simulink model "Fault_RLready_AC_Droop_four_Inverters"  (R2025a)
settings: Solver=ode4  StartTime=0.0  StopTime=15  MaxStep=1e-4  RelTol=1e-3
PreLoadFcn:
  | k_couple = 1;
  | k_power  = 0.0001;
  | k_corr   = 5;
InitFcn:
  | K1=1e-4;
libraries: spsThreePhaseSeriesRLCBranchLib x16, slpidlib x16, spsThreePhaseVIMeasurementLib x12, spsFirstOrderFilterLib x8, spsThreePhaseParallelRLCLoadLib x5, spsDCVoltageSourceLib x4, spsUniversalBridgeLib x4, simulink x4, MGLib x4, spsVoltageMeasurementLib x4, spsThreePhaseBreakerLib x1, spspowerguiLib x1
(part 1 of 4)
settings Model: SimulationMode=accelerator  Creator=Admin  LastModifiedBy=rks9560
settings SolverCC: AlgebraicLoopSolver=TrustRegion
settings OptimizationCC: ReuseModelBlockBuffer=off  EfficientMapNaN2IntZero=off
settings DebuggingCC: UnconnectedInputMsg=warning  UnconnectedOutputMsg=warning  UnconnectedLineMsg=warning  ArithmeticOperatorsInVariantConditions=warning
settings HardwareCC: TargetBitPerPointer=64.0  TargetBitPerSizeT=64.0  TargetBitPerPtrDiffT=64.0  TargetLongLongMode=on  TargetIntDivRoundTo=Zero  TargetEndianess=LittleEndian  TargetWordSize=64.0  TargetHWDeviceType=MATLAB Host  ProdEqTarget=off
settings ModelReferenceCC: EnableRefExpFcnMdlSchedulingChecks=on
settings SFSimCC: SimUseLocalCustomCode=off  CustomCodeUndefinedFunction=UseInterfaceOnly
settings RTWCC: GPUComputeCapability=3.5
settings CodeAppCC: MaxIdLength=128.0
settings GRTTargetCC: TargetLangStandard=C89/C90 (ANSI)  CombineOutputUpdateFcns=off  GRTInterface=on
settings SimscapeCC: SimscapeNormalizeSystem=off

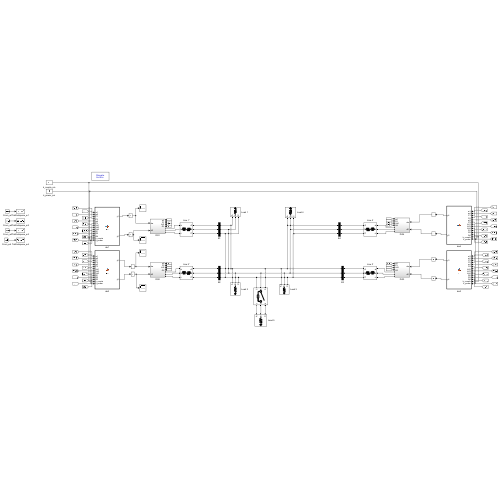
[thumbnail: Simulink's stored preview of the top-level diagram]
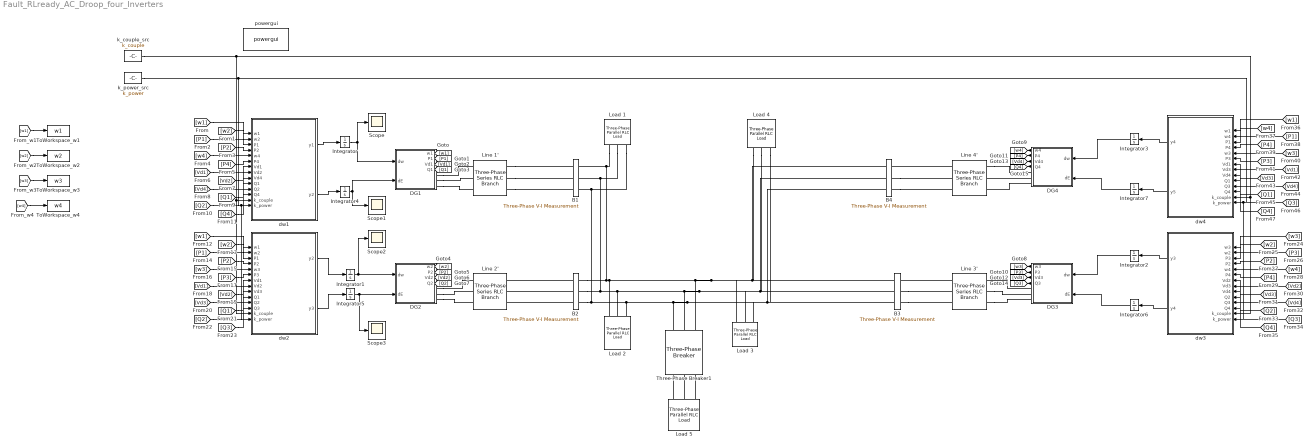
== system Fault_RLready_AC_Droop_four_Inverters ==
  B1 : spsThreePhaseVIMeasurementLib/Three-Phase V-I Measurement  VoltageMeasurement=phase-to-ground  SetLabelV=on  LabelV=VB1  Vpu=off  VpuLL=off  CurrentMeasurement=yes  SetLabelI=on  LabelI=IB1  Ipu=off  Pbase=100e6  Vbase=500e3  OutputType=Complex  PhasorSimulation=off  PSBequivalent=0
  B2 : spsThreePhaseVIMeasurementLib/Three-Phase V-I Measurement  VoltageMeasurement=phase-to-ground  SetLabelV=on  LabelV=VB2  Vpu=off  VpuLL=off  CurrentMeasurement=yes  SetLabelI=on  LabelI=IB2  Ipu=off  Pbase=100e6  Vbase=500e3  OutputType=Complex  PhasorSimulation=off  PSBequivalent=0
  B3 : spsThreePhaseVIMeasurementLib/Three-Phase V-I Measurement  VoltageMeasurement=phase-to-ground  SetLabelV=on  LabelV=VB3  Vpu=off  VpuLL=off  CurrentMeasurement=yes  SetLabelI=on  LabelI=IB3  Ipu=off  Pbase=100e6  Vbase=500e3  OutputType=Complex  PhasorSimulation=off  PSBequivalent=0
  B4 : spsThreePhaseVIMeasurementLib/Three-Phase V-I Measurement  VoltageMeasurement=phase-to-ground  SetLabelV=on  LabelV=VB4  Vpu=off  VpuLL=off  CurrentMeasurement=yes  SetLabelI=on  LabelI=IB4  Ipu=off  Pbase=100e6  Vbase=500e3  OutputType=Complex  PhasorSimulation=off  PSBequivalent=0
  DG1 : Subsystem
  DG2 : Subsystem
  DG3 : Subsystem
  DG4 : Subsystem
  Integrator{,1..7} (8 alike) : Integrator
  Line 1' : spsThreePhaseSeriesRLCBranchLib/Three-Phase Series RLC Branch  LConnTagsString=A|B|C  RConnTagsString=A|B|C  BranchType=RL  Resistance=0.07  Inductance=0.05e-2  Capacitance=1e-6  Measurements=None
  Line 2' : spsThreePhaseSeriesRLCBranchLib/Three-Phase Series RLC Branch  LConnTagsString=A|B|C  RConnTagsString=A|B|C  BranchType=RL  Resistance=0.07  Inductance=0.05e-2  Capacitance=1e-6  Measurements=None
  Line 3' : spsThreePhaseSeriesRLCBranchLib/Three-Phase Series RLC Branch  LConnTagsString=A|B|C  RConnTagsString=A|B|C  BranchType=RL  Resistance=0.01  Inductance=0.05e-2  Capacitance=1e-6  Measurements=None
  Line 4' : spsThreePhaseSeriesRLCBranchLib/Three-Phase Series RLC Branch  LConnTagsString=A|B|C  RConnTagsString=A|B|C  BranchType=RL  Resistance=0.07  Inductance=0.05e-2  Capacitance=1e-6  Measurements=None
  Load {1..4} (4 alike) : spsThreePhaseParallelRLCLoadLib/Three-Phase Parallel RLC Load  LConnTagsString=A|B|C  Configuration=Y (grounded)  NominalVoltage=415  Vabc=[1e3 1e3 1e3]  Vabcp=[1e3 1e3 1e3]  NominalFrequency=60  UnbalancedPower=off  ActivePower=5e3  InductivePower=0  CapacitivePower=0  Pabc=[10e3 9e3 11e3]  QLabc=[100 90 110]  QCabc=[100 90 110]  Pabcp=[10e3 9e3 11e3]  QLabcp=[100 90 110]  QCabcp=[100 90 110]  Measurements=None  LoadType=constant PQ
  Load 5 : spsThreePhaseParallelRLCLoadLib/Three-Phase Parallel RLC Load  LConnTagsString=A|B|C  Configuration=Y (grounded)  NominalVoltage=415  Vabc=[1e3 1e3 1e3]  Vabcp=[1e3 1e3 1e3]  NominalFrequency=60  UnbalancedPower=off  ActivePower=20e3  InductivePower=0  CapacitivePower=0  Pabc=[10e3 9e3 11e3]  QLabc=[100 90 110]  QCabc=[100 90 110]  Pabcp=[10e3 9e3 11e3]  QLabcp=[100 90 110]  QCabcp=[100 90 110]  Measurements=None  LoadType=constant PQ
  Scope{,1..3} (4 alike) : Scope
      Scope settings: ActiveDisplayYMinimum=-117.83448  ActiveDisplayYMaximum=1060.51036
      Scope1 settings: ActiveDisplayYMinimum=-75.78712  ActiveDisplayYMaximum=9.50958  DataLoggingVariableName=ScopeData2
      Scope2 settings: ActiveDisplayYMinimum=-0.02486  ActiveDisplayYMaximum=0.2237  DataLoggingVariableName=ScopeData3
      Scope3 settings: ActiveDisplayYMinimum=-0.00731  ActiveDisplayYMaximum=0.06583  DataLoggingVariableName=ScopeData4
  Three-Phase Breaker1 : spsThreePhaseBreakerLib/Three-Phase Breaker  InitialState=open  SwitchA=on  SwitchB=on  SwitchC=on  SwitchTimes=[6]  External=off  BreakerResistance=0.01  SnubberResistance=1e6  SnubberCapacitance=inf  Measurements=None
  ToWorkspace_w1 : ToWorkspace  VariableName=w1  SaveFormat=Structure With Time  SampleTime=-1
  ToWorkspace_w2 : ToWorkspace  VariableName=w2  SaveFormat=Structure With Time  SampleTime=-1
  ToWorkspace_w3 : ToWorkspace  VariableName=w3  SaveFormat=Structure With Time  SampleTime=-1
  ToWorkspace_w4 : ToWorkspace  VariableName=w4  SaveFormat=Structure With Time  SampleTime=-1
  dw1 : MATLAB Function  TreatAsAtomicUnit=on
  dw2 : MATLAB Function  TreatAsAtomicUnit=on
  dw3 : MATLAB Function  TreatAsAtomicUnit=on
  dw4 : MATLAB Function  TreatAsAtomicUnit=on
  k_couple_src : Constant  Value=k_couple
  k_power_src : Constant  Value=k_power
  powergui : spspowerguiLib/powergui  Priority=1  SimulationMode=Discrete  SampleTime=0.2e-5  frequency=60  Iterations=50  frequencyindice=0  Pbase=100e6  ErrMax=1e-4  UnitsV=kV  UnitsW=MW  buscounter=0  FunctionMessages=off  echomessages=off  EnableUseOfTLC=off  CurrentSourceSwitches=off  DisableSnubberDevices=off  DisableRonSwitches=off  DisableVfSwitches=off  DisplayEquations=off  AutomaticDiscreteSolvers=off  SolverType=Tustin/Backward Euler (TBE)  Interpol=off  ExternalGateDelay=off  methode=off  Ts=100  x0status=blocks  SPID=off  SwTol=0  HookPort=off  NonlinearTolerance=1e-4  nMaxIteration=100  ContinueOnMaxIteration=off  RestoreLinks=warning  ResistiveCurrentMeasurement=off  Frange=[0:2:500]  Ylog=off  Xlog=on  ShowGrid=off  save=off  variable=ZData  structure=0  ZoomFFT=off  StartTime=0.0  cycles=1  DisplayStyle=1  fundamental=60  FreqAxis=off  MaxFrequency=1000  frequencyindicesteady=1  RmsSteady=1  display=off
  wires:
  Integrator2/1 -> DG3/1(dw)
  Integrator3/1 -> DG4/1(dw)
  dw1/1(y1) -> Integrator/1
  dw2/1(y2) -> Integrator1/1
  dw4/1(y4) -> Integrator3/1
  dw3/1(y3) -> Integrator2/1
  dw1/2(y2) -> Integrator4/1
  dw2/2(y3) -> Integrator5/1
  dw3/2(y4) -> Integrator6/1
  Integrator6/1 -> DG3/2(dE)
  dw4/2(y5) -> Integrator7/1
  Integrator7/1 -> DG4/2(dE)
  DG4/3(Vd4) -> [Vd4]
  DG1/1(w1) -> [w1]
  DG1/2(P1) -> [P1]
  DG1/3(Vd1) -> [Vd1]
  DG1/4(Q1) -> [Q1]
  DG2/1(w2) -> [w2]
  DG2/2(P2) -> [P2]
  DG2/3(Vd2) -> [Vd2]
  DG2/4(Q2) -> [Q2]
  DG3/1(w3) -> [w3]
  DG4/1(w4) -> [w4]
  DG3/2(P3) -> [P3]
  DG4/2(P4) -> [P4]
  DG3/3(Vd3) -> [Vd3]
  DG3/4(Q3) -> [Q3]
  DG4/4(Q4) -> [Q4]
  Integrator/1 -> DG1/1(dw), Scope/1
  Integrator4/1 -> DG1/2(dE), Scope1/1
  Integrator1/1 -> DG2/1(dw), Scope2/1
  Integrator5/1 -> Scope3/1, DG2/2(dE)
  [w1] -> dw1/1(w1)
  [w2] -> dw1/2(w2)
  [P1] -> dw1/3(P1)
  [P2] -> dw1/4(P2)
  [w4] -> dw1/5(w4)
  [P4] -> dw1/6(P4)
  [Vd1] -> dw1/7(Vd1)
  [Vd2] -> dw1/8(Vd2)
  [Vd4] -> dw1/9(Vd4)
  [Q1] -> dw1/10(Q1)
  [Q2] -> dw1/11(Q2)
  [Q4] -> dw1/12(Q4)
  [w1] -> dw2/1(w1)
  [w2] -> dw2/2(w2)
  [P1] -> dw2/3(P1)
  [P2] -> dw2/4(P2)
  [w3] -> dw2/5(w3)
  [P3] -> dw2/6(P3)
  [Vd1] -> dw2/7(Vd1)
  [Vd2] -> dw2/8(Vd2)
  [Vd3] -> dw2/9(Vd3)
  [Q1] -> dw2/10(Q1)
  [Q2] -> dw2/11(Q2)
  [Q3] -> dw2/12(Q3)
  [w1] -> dw4/1(w1)
  [w4] -> dw4/2(w4)
  [P1] -> dw4/3(P1)
  [P4] -> dw4/4(P4)
  [w3] -> dw4/5(w3)
  [P3] -> dw4/6(P3)
  [Vd1] -> dw4/7(Vd1)
  [Vd3] -> dw4/8(Vd3)
  [Vd4] -> dw4/9(Vd4)
  [Q1] -> dw4/10(Q1)
  [Q3] -> dw4/11(Q3)
  [Q4] -> dw4/12(Q4)
  [w3] -> dw3/1(w3)
  [w2] -> dw3/2(w2)
  [P3] -> dw3/3(P3)
  [P2] -> dw3/4(P2)
  [w4] -> dw3/5(w4)
  [P4] -> dw3/6(P4)
  [Vd2] -> dw3/7(Vd2)
  [Vd3] -> dw3/8(Vd3)
  [Vd4] -> dw3/9(Vd4)
  [Q2] -> dw3/10(Q2)
  [Q3] -> dw3/11(Q3)
  [Q4] -> dw3/12(Q4)
  k_couple_src/1 -> dw4/13(k_couple), dw3/13(k_couple), dw1/13(k_couple), dw2/13(k_couple)
  k_power_src/1 -> dw3/14(k_power), dw4/14(k_power), dw1/14(k_power), dw2/14(k_power)
  [w1] -> ToWorkspace_w1/1
  [w2] -> ToWorkspace_w2/1
  [w3] -> ToWorkspace_w3/1
  [w4] -> ToWorkspace_w4/1
  connections:
  Line 1'/LConn3 -- B1/LConn3
  Line 1'/LConn1 -- B1/LConn1
  Line 1'/LConn2 -- B1/LConn2
  B2/LConn1 -- Line 2'/LConn1
  B2/LConn2 -- Line 2'/LConn2
  B2/LConn3 -- Line 2'/LConn3
  Line 3'/LConn1 -- B3/LConn1
  B3/LConn2 -- Line 3'/LConn2
  B3/LConn3 -- Line 3'/LConn3
  Line 4'/LConn1 -- B4/LConn1
  B4/LConn2 -- Line 4'/LConn2
  B4/LConn3 -- Line 4'/LConn3
  B2/RConn1 -- Three-Phase Breaker1/LConn1 -- B3/RConn1 -- B4/RConn1 -- Load 4/LConn1 -- Load 3/LConn1 -- Load 2/LConn1 -- Load 1/LConn1 -- B1/RConn1
  B2/RConn2 -- Three-Phase Breaker1/LConn2 -- B3/RConn2 -- B4/RConn2 -- Load 4/LConn2 -- Load 3/LConn2 -- Load 2/LConn2 -- Load 1/LConn2 -- B1/RConn2
  B2/RConn3 -- Three-Phase Breaker1/LConn3 -- B3/RConn3 -- B4/RConn3 -- Load 4/LConn3 -- Load 3/LConn3 -- Load 2/LConn3 -- Load 1/LConn3 -- B1/RConn3
  DG1/RConn1 -- Line 1'/RConn1
  DG1/RConn2 -- Line 1'/RConn2
  DG1/RConn3 -- Line 1'/RConn3
  DG2/RConn1 -- Line 2'/RConn1
  DG2/RConn2 -- Line 2'/RConn2
  DG2/RConn3 -- Line 2'/RConn3
  DG3/RConn1 -- Line 3'/RConn1
  Line 3'/RConn2 -- DG3/RConn2
  Line 3'/RConn3 -- DG3/RConn3
  Line 4'/RConn1 -- DG4/RConn1
  DG4/RConn2 -- Line 4'/RConn2
  DG4/RConn3 -- Line 4'/RConn3
  Load 5/LConn1 -- Three-Phase Breaker1/RConn3
  Load 5/LConn2 -- Three-Phase Breaker1/RConn2
  Load 5/LConn3 -- Three-Phase Breaker1/RConn1

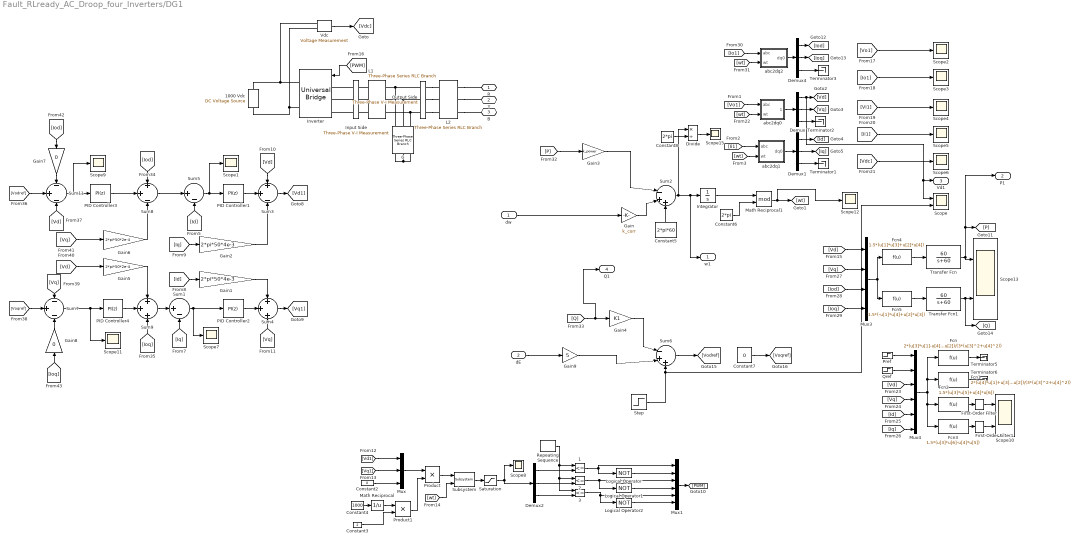
== system Fault_RLready_AC_Droop_four_Inverters/DG1 ==
  dw : Inport
  dE : Inport  Port=2
  1 : RelationalOperator  Operator=<=  OutDataTypeStr=boolean  RndMeth=Simplest  InputSameDT=off
  1000 Vdc : spsDCVoltageSourceLib/DC Voltage Source  Amplitude=1000  Measurements=None
  2 : RelationalOperator  Operator=<=  OutDataTypeStr=boolean  RndMeth=Simplest  InputSameDT=off
  3 : RelationalOperator  Operator=<=  OutDataTypeStr=boolean  RndMeth=Simplest  InputSameDT=off
  C : spsThreePhaseSeriesRLCBranchLib/Three-Phase Series RLC Branch  LConnTagsString=A|B|C  RConnTagsString=A|B|C  BranchType=RC  Resistance=5  Inductance=1e-3  Capacitance=2e-4  Measurements=None
  Constant2 : Constant  Value=0
  Constant3 : Constant  Value=2
  Constant4 : Constant  Value=1000
  Constant5 : Constant  Value=2*pi*60
  Constant6 : Constant  Value=2*pi
  Constant7 : Constant  Value=0
  Constant8 : Constant  Value=2*pi
  Demux{,1..2,4} (4 alike) : Demux  Outputs=3
  Divide : Product  Inputs=*/
  Fcn : Fcn  Expr=2*(u[3]*u[1]-u[4]*u[2])/(3*(u[3]^2+u[4]^2))
  Fcn1 : Fcn  Expr=2*(u[4]*u[1]+u[3]*u[2])/(3*(u[3]^2+u[4]^2))
  Fcn2 : Fcn  Expr=1.5*(u[3]*u[5]+u[4]*u[6])
  Fcn3 : Fcn  Expr=1.5*(u[3]*u[6]-u[4]*u[5])
  Fcn4 : Fcn  Expr=1.5*(u[1]*u[3]+u[2]*u[4])
  Fcn5 : Fcn  Expr=1.5*(-u[1]*u[4]+u[2]*u[3])
  First-Order Filter : spsFirstOrderFilterLib/First-Order Filter  FilterType=Lowpass  Tc=0.03  Ts=0  Initialize=on  Vac_Init=[0, 0, 60]  Vdc_Init=0  PlotResponse=off  FreqRange="[0,  200,  1]"
  First-Order Filter1 : spsFirstOrderFilterLib/First-Order Filter  FilterType=Lowpass  Tc=0.03  Ts=0  Initialize=on  Vac_Init=[0, 0, 60]  Vdc_Init=0  PlotResponse=off  FreqRange="[0,  200,  1]"
  Gain : Gain  Gain=k_corr
  Gain1 : Gain  Gain=2*pi*50*4e-3
  Gain2 : Gain  Gain=2*pi*50*4e-3
  Gain3 : Gain  Gain=k_power
  Gain4 : Gain  Gain=K1
  Gain5 : Gain  Gain=2*pi*50*2e-4
  Gain6 : Gain  Gain=2*pi*50*2e-4
  Gain7 : Gain  Gain=0
  Gain8 : Gain  Gain=0
  Gain9 : Gain  Gain=5
  Input Side : spsThreePhaseVIMeasurementLib/Three-Phase V-I Measurement  VoltageMeasurement=phase-to-ground  SetLabelV=on  LabelV=Vi1  Vpu=off  VpuLL=off  CurrentMeasurement=yes  SetLabelI=on  LabelI=Ii1  Ipu=off  Pbase=100e6  Vbase=500e3  OutputType=Complex  PhasorSimulation=off  PSBequivalent=0
  Integrator : Integrator
  Inverter : spsUniversalBridgeLib/Universal Bridge  Arms=3  SnubberResistance=1e5  SnubberCapacitance=inf  Device=Ideal Switches  Ron=1e-3  Lon=0  ForwardVoltages="[  0  0  ]"  ForwardVoltage=0  GTOparameters=[ 10e-6 , 20e-6 ]  IGBTparameters=[ 1e-6 , 2e-6 ]  Measurements=None  Measurements_2=None  converterType=Rectifier
  L1 : spsThreePhaseSeriesRLCBranchLib/Three-Phase Series RLC Branch  LConnTagsString=A|B|C  RConnTagsString=A|B|C  BranchType=RL  Resistance=0.1  Inductance=4e-3  Capacitance=1e-6  Measurements=None
  L2 : spsThreePhaseSeriesRLCBranchLib/Three-Phase Series RLC Branch  LConnTagsString=A|B|C  RConnTagsString=A|B|C  BranchType=RL  Resistance=0.03  Inductance=1e-3  Capacitance=1e-6  Measurements=None
  Logical Operator : Logic  Operator=NOT  IconShape=distinctive  AllPortsSameDT=off  OutDataTypeStr=boolean
  Logical Operator1 : Logic  Operator=NOT  IconShape=distinctive  AllPortsSameDT=off  OutDataTypeStr=boolean
  Logical Operator2 : Logic  Operator=NOT  IconShape=distinctive  AllPortsSameDT=off  OutDataTypeStr=boolean
  Math Reciprocal : Math  Operator=reciprocal  SignedPower=on
  Math Reciprocal1 : Math  Operator=mod  SignedPower=on
  Mux : Mux  Inputs=3
  Mux1 : Mux  Inputs=6
  Mux3 : Mux
  Mux4 : Mux  Inputs=6
  Output Side : spsThreePhaseVIMeasurementLib/Three-Phase V-I Measurement  VoltageMeasurement=phase-to-ground  SetLabelV=on  LabelV=Vo1  Vpu=off  VpuLL=off  CurrentMeasurement=yes  SetLabelI=on  LabelI=Io1  Ipu=off  Pbase=100e6  Vbase=500e3  OutputType=Complex  PhasorSimulation=off  PSBequivalent=0
  PID Controller1 : slpidlib/PID Controller  Controller=PI  Form=Parallel  TimeDomain=Discrete-time  UseExternalTs=off  SampleTime=-1  IntegratorMethod=Forward Euler  FilterMethod=Forward Euler  ControllerParametersSource=internal  P=4e-3/1e-4  I=0.1/1e-4  UseKiTs=off  D=0  UseExternalDerivativeSource=off  N=100  UseFilter=on  TunerSelectOption=Transfer Function Based (PID Tuner App)  InitialConditionSource=internal  InitialConditionForIntegrator=0  InitialConditionForFilter=0  DifferentiatorICPrevScaledInput=0  ExternalReset=none  TrackingMode=off  Kt=1  LimitOutput=off  SatLimitsSource=internal  UpperSaturationLimit=inf  LowerSaturationLimit=-inf  LinearizeAsGain=on  AntiWindupMode=none  Kb=1  LimitIntegrator=off  UpperIntegratorSaturationLimit=inf  LowerIntegratorSaturationLimit=-inf  POutMin=[]  POutMax=[]  IOutMin=[]  IOutMax=[]  DOutMin=[]  DOutMax=[]  NOutMin=[]  NOutMax=[]  SumOutMin=[]  SumOutMax=[]  SaturationOutMin=[]  SaturationOutMax=[]  PParamMin=[]  PParamMax=[]  IParamMin=[]  IParamMax=[]  DParamMin=[]  DParamMax=[]  NParamMin=[]  NParamMax=[]  KbParamMin=[]  KbParamMax=[]  KtParamMin=[]  KtParamMax=[]  KbOutMin=[]  KbOutMax=[]  KtOutMin=[]  KtOutMax=[]  IntegratorOutMin=[]  IntegratorOutMax=[]  FilterOutMin=[]  FilterOutMax=[]  SumI1OutMin=[]  SumI1OutMax=[]  SumI2OutMin=[]  SumI2OutMax=[]  SumI3OutMin=[]  SumI3OutMax=[]  SumI4OutMin=[]  SumI4OutMax=[]  SumDOutMin=[]  SumDOutMax=[]  DifferentiatorOutMin=[]  DifferentiatorOutMax=[]  FilterDiffOutCoefMin=[]  FilterDiffOutCoefMax=[]  ReciprocalOutMin=[]  ReciprocalOutMax=[]  SumDenOutMin=[]  SumDenOutMax=[]  SumNumOutMin=[]  SumNumOutMax=[]  DivideOutMin=[]  DivideOutMax=[]  UdiffTsProdOutMin=[]  UdiffTsProdOutMax=[]  NTsProdOutMin=[]  NTsProdOutMax=[]  UintegralTsProdOutMin=[]  UintegralTsProdOutMax=[]  UngainTsProdOutMin=[]  UngainTsProdOutMax=[]  ClampingZeroOutDataTypeStr=Inherit: Inherit via back propagation  ClampingZeroOutMin=[]  ClampingZeroOutMax=[]  FilterDenConstantOutDataTypeStr=Inherit: Inherit via back propagation  FilterDenConstantOutMin=[]  FilterDenConstantOutMax=[]  PCopyOutDataTypeStr=Inherit: Inherit via back propagation  PCopyOutMin=[]  PCopyOutMax=[]  NCopyOutDataTypeStr=Inherit: Inherit via back propagation  NCopyOutMin=[]  NCopyOutMax=[]  IntegratorContinuousStateAttributes=''  IntegratorStateMustResolveToSignalObject=off  IntegratorRTWStateStorageClass=Auto  FilterContinuousStateAttributes=''  FilterStateMustResolveToSignalObject=off  FilterRTWStateStorageClass=Auto  ParallelPVariant=InternalParameters  IdealPVariant=Disabled  IVariant=InternalParameters  DVariant=Disabled  IntegratorVariant=Discrete  SatVariant=Disabled  AWVariant=Passthrough  PCopyVariant=Disabled  TRVariant=Disabled  FdbkBlocksVariant=Forward  IdealPFdbkVariant=Disabled  SatFdbkVariant=Disabled  DerivativeFilterVariant=Disabled  NVariant=Disabled  NCopyVariant=Disabled_SignalSpec  FilterICVariant=Disabled  IntegratorICVariant=InternalICs  ExternalResetVariant=Disabled  TRSumVariant=Passthrough  SumFdbkVariant=Disabled  SumVariant=Sum_PI  TsampFilterVariant=InternalTs  TsampNgainVariant=Passthrough  TsampIntegralVariant=Disabled_SignalSpec  ExternalSaturationOutDataTypeStr=Inherit: Same as second input  DerivativeSourceVariant=Disabled  PreIntVariant=InternalPreInt
  PID Controller2 : slpidlib/PID Controller  Controller=PI  Form=Parallel  TimeDomain=Discrete-time  UseExternalTs=off  SampleTime=-1  IntegratorMethod=Forward Euler  FilterMethod=Forward Euler  ControllerParametersSource=internal  P=4e-3/1e-4  I=0.1/1e-4  UseKiTs=off  D=0  UseExternalDerivativeSource=off  N=100  UseFilter=on  TunerSelectOption=Transfer Function Based (PID Tuner App)  InitialConditionSource=internal  InitialConditionForIntegrator=0  InitialConditionForFilter=0  DifferentiatorICPrevScaledInput=0  ExternalReset=none  TrackingMode=off  Kt=1  LimitOutput=off  SatLimitsSource=internal  UpperSaturationLimit=inf  LowerSaturationLimit=-inf  LinearizeAsGain=on  AntiWindupMode=none  Kb=1  LimitIntegrator=off  UpperIntegratorSaturationLimit=inf  LowerIntegratorSaturationLimit=-inf  POutMin=[]  POutMax=[]  IOutMin=[]  IOutMax=[]  DOutMin=[]  DOutMax=[]  NOutMin=[]  NOutMax=[]  SumOutMin=[]  SumOutMax=[]  SaturationOutMin=[]  SaturationOutMax=[]  PParamMin=[]  PParamMax=[]  IParamMin=[]  IParamMax=[]  DParamMin=[]  DParamMax=[]  NParamMin=[]  NParamMax=[]  KbParamMin=[]  KbParamMax=[]  KtParamMin=[]  KtParamMax=[]  KbOutMin=[]  KbOutMax=[]  KtOutMin=[]  KtOutMax=[]  IntegratorOutMin=[]  IntegratorOutMax=[]  FilterOutMin=[]  FilterOutMax=[]  SumI1OutMin=[]  SumI1OutMax=[]  SumI2OutMin=[]  SumI2OutMax=[]  SumI3OutMin=[]  SumI3OutMax=[]  SumI4OutMin=[]  SumI4OutMax=[]  SumDOutMin=[]  SumDOutMax=[]  DifferentiatorOutMin=[]  DifferentiatorOutMax=[]  FilterDiffOutCoefMin=[]  FilterDiffOutCoefMax=[]  ReciprocalOutMin=[]  ReciprocalOutMax=[]  SumDenOutMin=[]  SumDenOutMax=[]  SumNumOutMin=[]  SumNumOutMax=[]  DivideOutMin=[]  DivideOutMax=[]  UdiffTsProdOutMin=[]  UdiffTsProdOutMax=[]  NTsProdOutMin=[]  NTsProdOutMax=[]  UintegralTsProdOutMin=[]  UintegralTsProdOutMax=[]  UngainTsProdOutMin=[]  UngainTsProdOutMax=[]  ClampingZeroOutDataTypeStr=Inherit: Inherit via back propagation  ClampingZeroOutMin=[]  ClampingZeroOutMax=[]  FilterDenConstantOutDataTypeStr=Inherit: Inherit via back propagation  FilterDenConstantOutMin=[]  FilterDenConstantOutMax=[]  PCopyOutDataTypeStr=Inherit: Inherit via back propagation  PCopyOutMin=[]  PCopyOutMax=[]  NCopyOutDataTypeStr=Inherit: Inherit via back propagation  NCopyOutMin=[]  NCopyOutMax=[]  IntegratorContinuousStateAttributes=''  IntegratorStateMustResolveToSignalObject=off  IntegratorRTWStateStorageClass=Auto  FilterContinuousStateAttributes=''  FilterStateMustResolveToSignalObject=off  FilterRTWStateStorageClass=Auto  ParallelPVariant=InternalParameters  IdealPVariant=Disabled  IVariant=InternalParameters  DVariant=Disabled  IntegratorVariant=Discrete  SatVariant=Disabled  AWVariant=Passthrough  PCopyVariant=Disabled  TRVariant=Disabled  FdbkBlocksVariant=Forward  IdealPFdbkVariant=Disabled  SatFdbkVariant=Disabled  DerivativeFilterVariant=Disabled  NVariant=Disabled  NCopyVariant=Disabled_SignalSpec  FilterICVariant=Disabled  IntegratorICVariant=InternalICs  ExternalResetVariant=Disabled  TRSumVariant=Passthrough  SumFdbkVariant=Disabled  SumVariant=Sum_PI  TsampFilterVariant=InternalTs  TsampNgainVariant=Passthrough  TsampIntegralVariant=Disabled_SignalSpec  ExternalSaturationOutDataTypeStr=Inherit: Same as second input  DerivativeSourceVariant=Disabled  PreIntVariant=InternalPreInt
  PID Controller3 : slpidlib/PID Controller  Controller=PI  Form=Parallel  TimeDomain=Discrete-time  UseExternalTs=off  SampleTime=-1  IntegratorMethod=Forward Euler  FilterMethod=Forward Euler  ControllerParametersSource=internal  P=2e-4/1e-3  I=5/1e-3  UseKiTs=off  D=0  UseExternalDerivativeSource=off  N=100  UseFilter=on  TunerSelectOption=Transfer Function Based (PID Tuner App)  InitialConditionSource=internal  InitialConditionForIntegrator=0  InitialConditionForFilter=0  DifferentiatorICPrevScaledInput=0  ExternalReset=none  TrackingMode=off  Kt=1  LimitOutput=off  SatLimitsSource=internal  UpperSaturationLimit=40  LowerSaturationLimit=-40  LinearizeAsGain=on  AntiWindupMode=back-calculation  Kb=1  LimitIntegrator=off  UpperIntegratorSaturationLimit=inf  LowerIntegratorSaturationLimit=-inf  POutMin=[]  POutMax=[]  IOutMin=[]  IOutMax=[]  DOutMin=[]  DOutMax=[]  NOutMin=[]  NOutMax=[]  SumOutMin=[]  SumOutMax=[]  SaturationOutMin=[]  SaturationOutMax=[]  PParamMin=[]  PParamMax=[]  IParamMin=[]  IParamMax=[]  DParamMin=[]  DParamMax=[]  NParamMin=[]  NParamMax=[]  KbParamMin=[]  KbParamMax=[]  KtParamMin=[]  KtParamMax=[]  KbOutMin=[]  KbOutMax=[]  KtOutMin=[]  KtOutMax=[]  IntegratorOutMin=[]  IntegratorOutMax=[]  FilterOutMin=[]  FilterOutMax=[]  SumI1OutMin=[]  SumI1OutMax=[]  SumI2OutMin=[]  SumI2OutMax=[]  SumI3OutMin=[]  SumI3OutMax=[]  SumI4OutMin=[]  SumI4OutMax=[]  SumDOutMin=[]  SumDOutMax=[]  DifferentiatorOutMin=[]  DifferentiatorOutMax=[]  FilterDiffOutCoefMin=[]  FilterDiffOutCoefMax=[]  ReciprocalOutMin=[]  ReciprocalOutMax=[]  SumDenOutMin=[]  SumDenOutMax=[]  SumNumOutMin=[]  SumNumOutMax=[]  DivideOutMin=[]  DivideOutMax=[]  UdiffTsProdOutMin=[]  UdiffTsProdOutMax=[]  NTsProdOutMin=[]  NTsProdOutMax=[]  UintegralTsProdOutMin=[]  UintegralTsProdOutMax=[]  UngainTsProdOutMin=[]  UngainTsProdOutMax=[]  ClampingZeroOutDataTypeStr=Inherit: Inherit via back propagation  ClampingZeroOutMin=[]  ClampingZeroOutMax=[]  FilterDenConstantOutDataTypeStr=Inherit: Inherit via back propagation  FilterDenConstantOutMin=[]  FilterDenConstantOutMax=[]  PCopyOutDataTypeStr=Inherit: Inherit via back propagation  PCopyOutMin=[]  PCopyOutMax=[]  NCopyOutDataTypeStr=Inherit: Inherit via back propagation  NCopyOutMin=[]  NCopyOutMax=[]  IntegratorContinuousStateAttributes=''  IntegratorStateMustResolveToSignalObject=off  IntegratorRTWStateStorageClass=Auto  FilterContinuousStateAttributes=''  FilterStateMustResolveToSignalObject=off  FilterRTWStateStorageClass=Auto  ParallelPVariant=InternalParameters  IdealPVariant=Disabled  IVariant=InternalParameters  DVariant=Disabled  IntegratorVariant=Discrete  SatVariant=Disabled  AWVariant=Passthrough  PCopyVariant=Disabled  TRVariant=Disabled  FdbkBlocksVariant=Forward  IdealPFdbkVariant=Disabled  SatFdbkVariant=Disabled  DerivativeFilterVariant=Disabled  NVariant=Disabled  NCopyVariant=Disabled_SignalSpec  FilterICVariant=Disabled  IntegratorICVariant=InternalICs  ExternalResetVariant=Disabled  TRSumVariant=Passthrough  SumFdbkVariant=Disabled  SumVariant=Sum_PI  TsampFilterVariant=InternalTs  TsampNgainVariant=Passthrough  TsampIntegralVariant=Disabled_SignalSpec  ExternalSaturationOutDataTypeStr=Inherit: Same as second input  DerivativeSourceVariant=Disabled  PreIntVariant=InternalPreInt
  PID Controller4 : slpidlib/PID Controller  Controller=PI  Form=Parallel  TimeDomain=Discrete-time  UseExternalTs=off  SampleTime=-1  IntegratorMethod=Forward Euler  FilterMethod=Forward Euler  ControllerParametersSource=internal  P=2e-4/1e-3  I=5/1e-3  UseKiTs=off  D=0  UseExternalDerivativeSource=off  N=100  UseFilter=on  TunerSelectOption=Transfer Function Based (PID Tuner App)  InitialConditionSource=internal  InitialConditionForIntegrator=0  InitialConditionForFilter=0  DifferentiatorICPrevScaledInput=0  ExternalReset=none  TrackingMode=off  Kt=1  LimitOutput=off  SatLimitsSource=internal  UpperSaturationLimit=40  LowerSaturationLimit=-40  LinearizeAsGain=on  AntiWindupMode=back-calculation  Kb=1  LimitIntegrator=off  UpperIntegratorSaturationLimit=inf  LowerIntegratorSaturationLimit=-inf  POutMin=[]  POutMax=[]  IOutMin=[]  IOutMax=[]  DOutMin=[]  DOutMax=[]  NOutMin=[]  NOutMax=[]  SumOutMin=[]  SumOutMax=[]  SaturationOutMin=[]  SaturationOutMax=[]  PParamMin=[]  PParamMax=[]  IParamMin=[]  IParamMax=[]  DParamMin=[]  DParamMax=[]  NParamMin=[]  NParamMax=[]  KbParamMin=[]  KbParamMax=[]  KtParamMin=[]  KtParamMax=[]  KbOutMin=[]  KbOutMax=[]  KtOutMin=[]  KtOutMax=[]  IntegratorOutMin=[]  IntegratorOutMax=[]  FilterOutMin=[]  FilterOutMax=[]  SumI1OutMin=[]  SumI1OutMax=[]  SumI2OutMin=[]  SumI2OutMax=[]  SumI3OutMin=[]  SumI3OutMax=[]  SumI4OutMin=[]  SumI4OutMax=[]  SumDOutMin=[]  SumDOutMax=[]  DifferentiatorOutMin=[]  DifferentiatorOutMax=[]  FilterDiffOutCoefMin=[]  FilterDiffOutCoefMax=[]  ReciprocalOutMin=[]  ReciprocalOutMax=[]  SumDenOutMin=[]  SumDenOutMax=[]  SumNumOutMin=[]  SumNumOutMax=[]  DivideOutMin=[]  DivideOutMax=[]  UdiffTsProdOutMin=[]  UdiffTsProdOutMax=[]  NTsProdOutMin=[]  NTsProdOutMax=[]  UintegralTsProdOutMin=[]  UintegralTsProdOutMax=[]  UngainTsProdOutMin=[]  UngainTsProdOutMax=[]  ClampingZeroOutDataTypeStr=Inherit: Inherit via back propagation  ClampingZeroOutMin=[]  ClampingZeroOutMax=[]  FilterDenConstantOutDataTypeStr=Inherit: Inherit via back propagation  FilterDenConstantOutMin=[]  FilterDenConstantOutMax=[]  PCopyOutDataTypeStr=Inherit: Inherit via back propagation  PCopyOutMin=[]  PCopyOutMax=[]  NCopyOutDataTypeStr=Inherit: Inherit via back propagation  NCopyOutMin=[]  NCopyOutMax=[]  IntegratorContinuousStateAttributes=''  IntegratorStateMustResolveToSignalObject=off  IntegratorRTWStateStorageClass=Auto  FilterContinuousStateAttributes=''  FilterStateMustResolveToSignalObject=off  FilterRTWStateStorageClass=Auto  ParallelPVariant=InternalParameters  IdealPVariant=Disabled  IVariant=InternalParameters  DVariant=Disabled  IntegratorVariant=Discrete  SatVariant=Disabled  AWVariant=Passthrough  PCopyVariant=Disabled  TRVariant=Disabled  FdbkBlocksVariant=Forward  IdealPFdbkVariant=Disabled  SatFdbkVariant=Disabled  DerivativeFilterVariant=Disabled  NVariant=Disabled  NCopyVariant=Disabled_SignalSpec  FilterICVariant=Disabled  IntegratorICVariant=InternalICs  ExternalResetVariant=Disabled  TRSumVariant=Passthrough  SumFdbkVariant=Disabled  SumVariant=Sum_PI  TsampFilterVariant=InternalTs  TsampNgainVariant=Passthrough  TsampIntegralVariant=Disabled_SignalSpec  ExternalSaturationOutDataTypeStr=Inherit: Same as second input  DerivativeSourceVariant=Disabled  PreIntVariant=InternalPreInt
  Pref : Step  Time=10  Before=10000  After=15000  SampleTime=0
  Product : Product
  Product1 : Product
  Qref : Step  Time=10  Before=54.1077  After=400  SampleTime=0
  Repeating Sequence : simulink/Sources/Repeating Sequence  rep_seq_t=[0 0.25 .5 0.75 1]/10000  rep_seq_y=[0 +1 0 -1 0]
  Saturation : Saturate  UpperLimit=1  LowerLimit=-1
  Scope : Scope  NumInputPorts=2
      settings: ActiveDisplayYMinimum=-69.98007  ActiveDisplayYMaximum=629.82061  DataLoggingVariableName=V1
  Scope{1..9,11..12,15} (12 alike) : Scope
      Scope1 settings: ActiveDisplayYMinimum=-180.21885  ActiveDisplayYMaximum=213.91205
      Scope11 settings: ActiveDisplayYMinimum=-618.03777  ActiveDisplayYMaximum=687.74246
      Scope12 settings: ActiveDisplayYMinimum=-0.54674  ActiveDisplayYMaximum=6.66504  DataLoggingVariableName=ScopeData3
      Scope15 settings: ActiveDisplayYMinimum=59.702436312097646  ActiveDisplayYMaximum=60.033152452888437  DataLoggingVariableName=ScopeData2
      Scope2 settings: ActiveDisplayYMinimum=-666.15088  ActiveDisplayYMaximum=514.3237  DataLoggingVariableName=ScopeData5
      Scope3 settings: ActiveDisplayYMinimum=-218.09311  ActiveDisplayYMaximum=218.08761  DataLoggingVariableName=I
      Scope4 settings: ActiveDisplayYMinimum=-833.41339  ActiveDisplayYMaximum=833.42189  DataLoggingVariableName=ScopeData7
      Scope5 settings: ActiveDisplayYMinimum=-59.12258  ActiveDisplayYMaximum=51.28632  DataLoggingVariableName=ScopeData8
      Scope6 settings: ActiveDisplayYMinimum=600  ActiveDisplayYMaximum=800  DataLoggingVariableName=ScopeData9
      Scope7 settings: ActiveDisplayYMinimum=-3.91022  ActiveDisplayYMaximum=6.31766  DataLoggingVariableName=ScopeData2
      Scope8 settings: ActiveDisplayYMinimum=-1.25  ActiveDisplayYMaximum=1.25  DataLoggingVariableName=ScopeData3
      Scope9 settings: ActiveDisplayYMinimum=-290.97325  ActiveDisplayYMaximum=408.82601  DataLoggingVariableName=ScopeData2
  Scope10 : Scope  NumInputPorts=2
      settings: ActiveDisplayYMinimum=-89498.22819  ActiveDisplayYMaximum=161141.30686  DataLoggingVariableName=ScopeData10
  Scope13 : Scope  NumInputPorts=2
      settings: ActiveDisplayYMinimum=-6615.9612931220372  ActiveDisplayYMaximum=59543.6474527404  DataLoggingVariableName=ScopeData4
  Step : Step  Time=0.5  Before=338.8460811  After=338.8460811  SampleTime=0
  Subsystem : MGLib/Subsystem  Power=Power Variant  dq=q-axis leads d-axis  Alignment=90 deg. behind a-phase axis
  Sum1 : Sum  Inputs=|+-
  Sum11 : Sum  Inputs=-|+|-
  Sum2 : Sum  Inputs=|-++
  Sum3 : Sum  Inputs=+|+|-
  Sum4 : Sum  Inputs=+|+|+
  Sum5 : Sum  Inputs=|+-
  Sum6 : Sum  Inputs=|-++
  Sum7 : Sum  Inputs=-|+|-
  Sum8 : Sum  Inputs=+|+|-
  Sum9 : Sum  Inputs=+|+|+
  Terminator{1..3,5..6} (5 alike) : Terminator
  Transfer Fcn : TransferFcn  Numerator=60  Denominator=[1 60]
  Transfer Fcn1 : TransferFcn  Numerator=60  Denominator=[1 60]
  Vdc : spsVoltageMeasurementLib/Voltage Measurement  PhasorSimulation=off  OutputType=Complex  PSBequivalent=0
  abc2dq0 : Subsystem  mask(abc to dq0 Transformation){Power=Power Variant, dq=q-axis leads d-axis, Alignment=90 deg. behind a-phase axis}
      mask prompts: Power "Power Variant/Invariant"; dq "d-q Axes Arrangement"; Alignment "Rotating frame alignment at wt=0"
      mask init:
      | str=cat(2);
      | if Power==1
      |     set_param(str,'Power','Power Variant Transform');
      | else
      |     set_param(str,'Power','Power Invariant Transform');
      | end
      | 
      | str1=cat(2);
      | if dq==1
      |     set_param(str1,'dq','q-axis leads d-axis');
      | else
      |     set_param(str1,'dq','q-axis lags d-axis');
      | end
      | 
      | str1=cat(2);
      | if Alignment==1
      |     set_param(str1,'Alignment','Along a-phase axis');
      | else
      |     set_param(str1,'Alignment','90 deg. behind a-phase axis');
      | end
      mask TypeOptions Power: Power Variant | Power Invariant
      mask TypeOptions dq: q-axis leads d-axis | q-axis lags d-axis
      mask TypeOptions Alignment: Along a-phase axis | 90 deg. behind a-phase axis
      mask Display:
      | plot([0 1], [0,1])
      | port_label('input', 1, 'abc')
      | port_label('input', 2, 'wt')
      | port_label('output', 1, 'dq0')
  abc2dq1 : Subsystem  mask(abc to dq0 Transformation){Power=Power Variant, dq=q-axis leads d-axis, Alignment=90 deg. behind a-phase axis}
      mask prompts: Power "Power Variant/Invariant"; dq "d-q Axes Arrangement"; Alignment "Rotating frame alignment at wt=0"
      mask init: same as Fault_RLready_AC_Droop_four_Inverters/DG1/abc2dq0
      mask TypeOptions Power: Power Variant | Power Invariant
      mask TypeOptions dq: q-axis leads d-axis | q-axis lags d-axis
      mask TypeOptions Alignment: Along a-phase axis | 90 deg. behind a-phase axis
      mask Display:
      | plot([0 1], [0,1])
      | port_label('input', 1, 'abc')
      | port_label('input', 2, 'wt')
      | port_label('output', 1, 'dq0')
  abc2dq2 : Subsystem  mask(abc to dq0 Transformation){Power=Power Variant, dq=q-axis leads d-axis, Alignment=90 deg. behind a-phase axis}
      mask prompts: Power "Power Variant/Invariant"; dq "d-q Axes Arrangement"; Alignment "Rotating frame alignment at wt=0"
      mask init: same as Fault_RLready_AC_Droop_four_Inverters/DG1/abc2dq0
      mask TypeOptions Power: Power Variant | Power Invariant
      mask TypeOptions dq: q-axis leads d-axis | q-axis lags d-axis
      mask TypeOptions Alignment: Along a-phase axis | 90 deg. behind a-phase axis
      mask Display:
      | plot([0 1], [0,1])
      | port_label('input', 1, 'abc')
      | port_label('input', 2, 'wt')
      | port_label('output', 1, 'dq0')
  R : PMIOPort  Side=Right
  Y : PMIOPort  Port=2  Side=Right
  B : PMIOPort  Port=3  Side=Right
  w1 : Outport  VectorParamsAs1DForOutWhenUnconnected=off
  P1 : Outport  Port=2  VectorParamsAs1DForOutWhenUnconnected=off
  Vd1 : Outport  Port=3  VectorParamsAs1DForOutWhenUnconnected=off
  Q1 : Outport  Port=4  VectorParamsAs1DForOutWhenUnconnected=off
  wires:
  Vdc/1 -> [Vdc]
  Fcn/1 -> Terminator5/1
  [Iod] -> Mux3/3
  [Vd] -> Mux3/1
  [Vq] -> Mux3/2
  [Vq] -> Mux4/4
  [Iq] -> Mux4/6
  Fcn1/1 -> Terminator6/1
  Pref/1 -> Mux4/1
  [Id] -> Mux4/5
  Mux4/1 -> Fcn2/1, Fcn3/1, Fcn1/1, Fcn/1
  Fcn2/1 -> First-Order Filter/1
  [Vd] -> Mux4/3
  First-Order Filter/1 -> Scope10/1
  [Ioq] -> Mux3/4
  First-Order Filter1/1 -> Scope10/2
  Qref/1 -> Mux4/2
  Fcn3/1 -> First-Order Filter1/1
  1/1 -> Mux1/1, Logical Operator/1
  Demux2/1 -> 1/2
  Demux2/2 -> 2/2
  Repeating Sequence/1 -> 3/1, 2/1, 1/1
  Saturation/1 -> Demux2/1, Scope8/1
  [Vq] -> Sum4/3
  Mux1/1 -> [PWM]
  [Iq] -> Gain2/1
  [Id] -> Gain1/1
  Sum3/1 -> [Vd1]
  Demux2/3 -> 3/2
  Mux/1 -> Product/1
  Sum4/1 -> [Vq1]
  Logical Operator2/1 -> Mux1/6
  Sum5/1 -> Scope1/1, PID Controller1/1
  [Iq] -> Sum1/2
  PID Controller1/1 -> Sum3/2
  Logical Operator1/1 -> Mux1/4
  Math Reciprocal/1 -> Product1/1
  3/1 -> Logical Operator2/1, Mux1/5
  Constant3/1 -> Product1/2
  [wt] -> Subsystem/2
  Subsystem/1 -> Saturation/1
  [Vd] -> Sum3/1
  [Vq1] -> Mux/2
  Constant2/1 -> Mux/3
  Gain1/1 -> Sum4/1
  Logical Operator/1 -> Mux1/2
  [Vd1] -> Mux/1
  2/1 -> Logical Operator1/1, Mux1/3
  Product1/1 -> Product/2
  Product/1 -> Subsystem/1
  [Id] -> Sum5/2
  Sum1/1 -> Scope7/1, PID Controller2/1
  Constant4/1 -> Math Reciprocal/1
  Gain2/1 -> Sum3/3
  PID Controller2/1 -> Sum4/2
  Demux1/3 -> Terminator1/1
  Demux/2 -> [Vq]
  Demux4/3 -> Terminator3/1
  Demux4/1 -> [Iod]
  abc2dq0/1(dq0) -> Demux/1
  Demux4/2 -> [Ioq]
  [Vo1] -> Scope2/1
  Demux/3 -> Terminator2/1
  Demux1/1 -> [Id]
  [Io1] -> abc2dq2/1(abc)
  [Vdc] -> Scope6/1
  [Vi1] -> Scope4/1
  abc2dq2/1(dq0) -> Demux4/1
  Demux1/2 -> [Iq]
  [Ii1] -> abc2dq1/1(abc)
  [Vo1] -> abc2dq0/1(abc)
  [Io1] -> Scope3/1
  [Ii1] -> Scope5/1
  Demux/1 -> Vd1/1, Scope/1, [Vd]
  abc2dq1/1(dq0) -> Demux1/1
  [PWM] -> Inverter/1
  [wt] -> abc2dq1/2(wt)
  [wt] -> abc2dq0/2(wt)
  [wt] -> abc2dq2/2(wt)
  Sum8/1 -> Sum5/1
  [P] -> Gain3/1
  Gain3/1 -> Sum2/1
  [Q] -> Q1/1, Gain4/1
  Gain4/1 -> Sum6/1
  Step/1 -> Sum6/3, Scope/2
  Sum2/1 -> Divide/1, w1/1, Integrator/1
  Integrator/1 -> Math Reciprocal1/1
  Constant6/1 -> Math Reciprocal1/2
  Math Reciprocal1/1 -> Scope12/1, [wt]
  Sum6/1 -> [Vodref]
  Constant7/1 -> [Voqref]
  [Vodref] -> Sum11/2
  [Vd] -> Sum11/3
  [Voqref] -> Sum7/2
  Gain5/1 -> Sum9/1
  Gain6/1 -> Sum8/3
  [Vd] -> Gain5/1
  [Ioq] -> Sum9/3
  [Vq] -> Gain6/1
  [Iod] -> Sum8/1
  Transfer Fcn1/1 -> [Q], Scope13/2
  Fcn5/1 -> Transfer Fcn1/1
  Fcn4/1 -> Transfer Fcn/1
  Transfer Fcn/1 -> Scope13/1, P1/1, [P]
  Mux3/1 -> Fcn4/1, Fcn5/1
  Divide/1 -> Scope15/1
  Constant8/1 -> Divide/2
  [Iod] -> Gain7/1
  Gain7/1 -> Sum11/1
  [Vq] -> Sum7/1
  [Ioq] -> Gain8/1
  Gain8/1 -> Sum7/3
  PID Controller3/1 -> Sum8/2
  PID Controller4/1 -> Sum9/2
  Sum9/1 -> Sum1/1
  Sum11/1 -> PID Controller3/1, Scope9/1
  Sum7/1 -> PID Controller4/1, Scope11/1
  Constant5/1 -> Sum2/3
  Gain/1 -> Sum2/2
  dw/1 -> Gain/1
  dE/1 -> Gain9/1
  Gain9/1 -> Sum6/2
  connections:
  C/LConn1 -- Output Side/LConn1 -- L1/RConn1
  C/LConn3 -- Output Side/LConn3 -- L1/RConn3
  C/LConn2 -- Output Side/LConn2 -- L1/RConn2
  Inverter/RConn1 -- 1000 Vdc/RConn1 -- Vdc/LConn1
  L1/LConn2 -- Input Side/RConn2
  L1/LConn1 -- Input Side/RConn1
  Inverter/RConn2 -- Vdc/LConn2 -- 1000 Vdc/LConn1
  Input Side/LConn1 -- Inverter/LConn1
  Input Side/LConn3 -- Inverter/LConn3
  L1/LConn3 -- Input Side/RConn3
  Input Side/LConn2 -- Inverter/LConn2
  C/RConn1 -- C/RConn3 -- C/RConn2
  L2/RConn1 -- R/RConn1
  L2/RConn2 -- Y/RConn1
  L2/RConn3 -- B/RConn1
  Output Side/RConn1 -- L2/LConn1
  Output Side/RConn2 -- L2/LConn2
  Output Side/RConn3 -- L2/LConn3
